simulink model "heatdrive_ecc_coupled_se21"  (R2025b)
settings: Solver=ode23t  StartTime=0.0  StopTime=10  FixedStep=0.1  MaxStep=0.4  RelTol=1e-2  AbsTol=1e-3
values from neighbouring files (symbols this model uses):
  cold_load_heat_W = 0.0    (= 0)    [Build_Simulink_Exchange_Params.m]
  cold_load_T_init = get_stage_field(stage_config, 'cold_load_T_in', get_stage_field(stage_config,          'chip_T_in', get_option_field(exchange_options, 'cold_load_T_init', get_option_field(exchange_options, 'chip_T_init', 293.0))))    [Build_Simulink_Exchange_Params.m]    (also in Create_Simulink_Exchange_Runtime.m = get_option_field(options, 'cold_load_T_init',          get_o)
  cold_sink_T_init = get_stage_field(stage_config, 'cold_sink_T_in', get_option_field(exchange_options, 'cold_sink_T_init', 293.0))    [Build_Simulink_Exchange_Params.m]    (also in Create_Simulink_Exchange_Runtime.m = get_option_field(options, 'cold_sink_T_init', ambient_T_init)
  hot_sink_T_init = get_stage_field(stage_config, 'hot_sink_T_in', get_option_field(exchange_options, 'hot_sink_T_init', 293.0))    [Build_Simulink_Exchange_Params.m]    (also in Create_Simulink_Exchange_Runtime.m = get_option_field(options, 'hot_sink_T_init', ambient_T_init))
  mdot_cooldown_source_kgps = mdot_target_kgps    [Build_Simulink_Exchange_Params.m]
  mdot_hold_source_kgps = mdot_target_kgps    [Build_Simulink_Exchange_Params.m]
  pressure_pi_bias_MPa = pressure_pi_dp_guess_MPa    [Build_Simulink_Exchange_Params.m]
  pressure_pi_error_filter_tau_s = max(get_option_field(exchange_options, 'pressure_pi_error_filter_tau_s', 0.002), 1.0e-5)    [Build_Simulink_Exchange_Params.m]
  pressure_pi_error_normalization_gain_kgps_inv = 1.0    (= 1)    [Build_Simulink_Exchange_Params.m]
  pressure_pi_max_MPa = pressure_pi_dp_guess_MPa + pressure_pi_margin_MPa    [Build_Simulink_Exchange_Params.m]
  shex_sink_T_init = get_option_field(exchange_options, 'shex_sink_T_init', hot_sink_T_init)    [Build_Simulink_Exchange_Params.m]
undefined symbols (not defined in the file or in its folder): constitutive_sample_time_s, constitutive_state21_initial, se_constitutive_T21_initial, se_pressure_integrator_max_MPa, se_pressure_pi_ki_MPa_per_kgps_s, se_pressure_pi_kp_MPa_per_kgps, se_pressure_pi_min_MPa, se_solver_T_init_21_internal, se_stage2_pressure_integrator_min_MPa, se_stage4_pressure_integrator_min_MPa, sma_constitutive_T21_initial, sma_mdot_stage1_source_kgps, sma_mdot_stage3_source_kgps, sma_pressure_integrator_max_MPa, sma_pressure_integrator_min_MPa, sma_pressure_pi_ki_MPa_per_kgps_s, sma_pressure_pi_kp_MPa_per_kgps, sma_pressure_pi_min_MPa, sma_solver_T_init_21_internal
libraries: fl_lib x484, nesl_utility x232, SimscapeFluids_lib x20
(part 2 of 8)

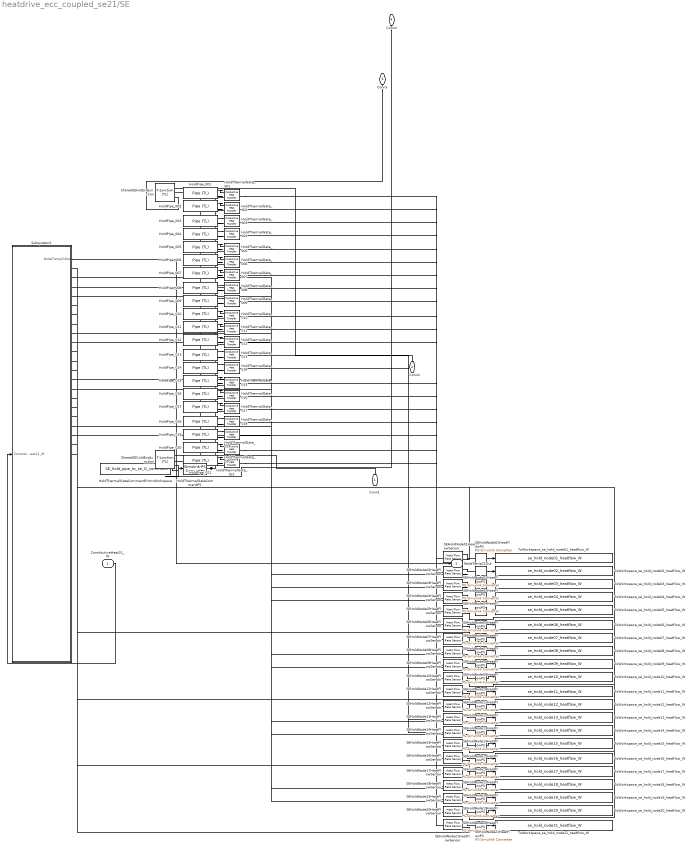
== system heatdrive_ecc_coupled_se21/SE ==
  ConstitutiveHeat21_W : Inport
  HoldPipe_001 : fl_lib/Thermal Liquid/Elements/Pipe (TL)  length=se_article_pipe_segment_l m  area=se_article_pipe_fa m^2  Dh=se_article_pipe_Dh m  length_add=0 m  roughness=15e-6 m  Re_lam=2000  Re_tur=4000  shape_factor=64  Nu_lam=se_article_Nu  dynamic_compressibility=false  inertia=false  p0=1 MPa  T0=se_hold_fluid_T_init K  mdot0=0 kg/s  p_nominal=1 MPa  T_nominal=293.15 K
  HoldPipe_002 : fl_lib/Thermal Liquid/Elements/Pipe (TL)  length=se_article_pipe_segment_l m  area=se_article_pipe_fa m^2  Dh=se_article_pipe_Dh m  length_add=0 m  roughness=15e-6 m  Re_lam=2000  Re_tur=4000  shape_factor=64  Nu_lam=se_article_Nu  dynamic_compressibility=false  inertia=false  p0=1 MPa  T0=se_hold_fluid_T_init K  mdot0=0 kg/s  p_nominal=1 MPa  T_nominal=293.15 K
  HoldPipe_003 : fl_lib/Thermal Liquid/Elements/Pipe (TL)  length=se_article_pipe_segment_l m  area=se_article_pipe_fa m^2  Dh=se_article_pipe_Dh m  length_add=0 m  roughness=15e-6 m  Re_lam=2000  Re_tur=4000  shape_factor=64  Nu_lam=se_article_Nu  dynamic_compressibility=false  inertia=false  p0=1 MPa  T0=se_hold_fluid_T_init K  mdot0=0 kg/s  p_nominal=1 MPa  T_nominal=293.15 K
  HoldPipe_004 : fl_lib/Thermal Liquid/Elements/Pipe (TL)  length=se_article_pipe_segment_l m  area=se_article_pipe_fa m^2  Dh=se_article_pipe_Dh m  length_add=0 m  roughness=15e-6 m  Re_lam=2000  Re_tur=4000  shape_factor=64  Nu_lam=se_article_Nu  dynamic_compressibility=false  inertia=false  p0=1 MPa  T0=se_hold_fluid_T_init K  mdot0=0 kg/s  p_nominal=1 MPa  T_nominal=293.15 K
  HoldPipe_005 : fl_lib/Thermal Liquid/Elements/Pipe (TL)  length=se_article_pipe_segment_l m  area=se_article_pipe_fa m^2  Dh=se_article_pipe_Dh m  length_add=0 m  roughness=15e-6 m  Re_lam=2000  Re_tur=4000  shape_factor=64  Nu_lam=se_article_Nu  dynamic_compressibility=false  inertia=false  p0=1 MPa  T0=se_hold_fluid_T_init K  mdot0=0 kg/s  p_nominal=1 MPa  T_nominal=293.15 K
  HoldPipe_006 : fl_lib/Thermal Liquid/Elements/Pipe (TL)  length=se_article_pipe_segment_l m  area=se_article_pipe_fa m^2  Dh=se_article_pipe_Dh m  length_add=0 m  roughness=15e-6 m  Re_lam=2000  Re_tur=4000  shape_factor=64  Nu_lam=se_article_Nu  dynamic_compressibility=false  inertia=false  p0=1 MPa  T0=se_hold_fluid_T_init K  mdot0=0 kg/s  p_nominal=1 MPa  T_nominal=293.15 K
  HoldPipe_007 : fl_lib/Thermal Liquid/Elements/Pipe (TL)  length=se_article_pipe_segment_l m  area=se_article_pipe_fa m^2  Dh=se_article_pipe_Dh m  length_add=0 m  roughness=15e-6 m  Re_lam=2000  Re_tur=4000  shape_factor=64  Nu_lam=se_article_Nu  dynamic_compressibility=false  inertia=false  p0=1 MPa  T0=se_hold_fluid_T_init K  mdot0=0 kg/s  p_nominal=1 MPa  T_nominal=293.15 K
  HoldPipe_008 : fl_lib/Thermal Liquid/Elements/Pipe (TL)  length=se_article_pipe_segment_l m  area=se_article_pipe_fa m^2  Dh=se_article_pipe_Dh m  length_add=0 m  roughness=15e-6 m  Re_lam=2000  Re_tur=4000  shape_factor=64  Nu_lam=se_article_Nu  dynamic_compressibility=false  inertia=false  p0=1 MPa  T0=se_hold_fluid_T_init K  mdot0=0 kg/s  p_nominal=1 MPa  T_nominal=293.15 K
  HoldPipe_009 : fl_lib/Thermal Liquid/Elements/Pipe (TL)  length=se_article_pipe_segment_l m  area=se_article_pipe_fa m^2  Dh=se_article_pipe_Dh m  length_add=0 m  roughness=15e-6 m  Re_lam=2000  Re_tur=4000  shape_factor=64  Nu_lam=se_article_Nu  dynamic_compressibility=false  inertia=false  p0=1 MPa  T0=se_hold_fluid_T_init K  mdot0=0 kg/s  p_nominal=1 MPa  T_nominal=293.15 K
  HoldPipe_010 : fl_lib/Thermal Liquid/Elements/Pipe (TL)  length=se_article_pipe_segment_l m  area=se_article_pipe_fa m^2  Dh=se_article_pipe_Dh m  length_add=0 m  roughness=15e-6 m  Re_lam=2000  Re_tur=4000  shape_factor=64  Nu_lam=se_article_Nu  dynamic_compressibility=false  inertia=false  p0=1 MPa  T0=se_hold_fluid_T_init K  mdot0=0 kg/s  p_nominal=1 MPa  T_nominal=293.15 K
  HoldPipe_011 : fl_lib/Thermal Liquid/Elements/Pipe (TL)  length=se_article_pipe_segment_l m  area=se_article_pipe_fa m^2  Dh=se_article_pipe_Dh m  length_add=0 m  roughness=15e-6 m  Re_lam=2000  Re_tur=4000  shape_factor=64  Nu_lam=se_article_Nu  dynamic_compressibility=false  inertia=false  p0=1 MPa  T0=se_hold_fluid_T_init K  mdot0=0 kg/s  p_nominal=1 MPa  T_nominal=293.15 K
  HoldPipe_012 : fl_lib/Thermal Liquid/Elements/Pipe (TL)  length=se_article_pipe_segment_l m  area=se_article_pipe_fa m^2  Dh=se_article_pipe_Dh m  length_add=0 m  roughness=15e-6 m  Re_lam=2000  Re_tur=4000  shape_factor=64  Nu_lam=se_article_Nu  dynamic_compressibility=false  inertia=false  p0=1 MPa  T0=se_hold_fluid_T_init K  mdot0=0 kg/s  p_nominal=1 MPa  T_nominal=293.15 K
  HoldPipe_013 : fl_lib/Thermal Liquid/Elements/Pipe (TL)  length=se_article_pipe_segment_l m  area=se_article_pipe_fa m^2  Dh=se_article_pipe_Dh m  length_add=0 m  roughness=15e-6 m  Re_lam=2000  Re_tur=4000  shape_factor=64  Nu_lam=se_article_Nu  dynamic_compressibility=false  inertia=false  p0=1 MPa  T0=se_hold_fluid_T_init K  mdot0=0 kg/s  p_nominal=1 MPa  T_nominal=293.15 K
  HoldPipe_014 : fl_lib/Thermal Liquid/Elements/Pipe (TL)  length=se_article_pipe_segment_l m  area=se_article_pipe_fa m^2  Dh=se_article_pipe_Dh m  length_add=0 m  roughness=15e-6 m  Re_lam=2000  Re_tur=4000  shape_factor=64  Nu_lam=se_article_Nu  dynamic_compressibility=false  inertia=false  p0=1 MPa  T0=se_hold_fluid_T_init K  mdot0=0 kg/s  p_nominal=1 MPa  T_nominal=293.15 K
  HoldPipe_015 : fl_lib/Thermal Liquid/Elements/Pipe (TL)  length=se_article_pipe_segment_l m  area=se_article_pipe_fa m^2  Dh=se_article_pipe_Dh m  length_add=0 m  roughness=15e-6 m  Re_lam=2000  Re_tur=4000  shape_factor=64  Nu_lam=se_article_Nu  dynamic_compressibility=false  inertia=false  p0=1 MPa  T0=se_hold_fluid_T_init K  mdot0=0 kg/s  p_nominal=1 MPa  T_nominal=293.15 K
  HoldPipe_016 : fl_lib/Thermal Liquid/Elements/Pipe (TL)  length=se_article_pipe_segment_l m  area=se_article_pipe_fa m^2  Dh=se_article_pipe_Dh m  length_add=0 m  roughness=15e-6 m  Re_lam=2000  Re_tur=4000  shape_factor=64  Nu_lam=se_article_Nu  dynamic_compressibility=false  inertia=false  p0=1 MPa  T0=se_hold_fluid_T_init K  mdot0=0 kg/s  p_nominal=1 MPa  T_nominal=293.15 K
  HoldPipe_017 : fl_lib/Thermal Liquid/Elements/Pipe (TL)  length=se_article_pipe_segment_l m  area=se_article_pipe_fa m^2  Dh=se_article_pipe_Dh m  length_add=0 m  roughness=15e-6 m  Re_lam=2000  Re_tur=4000  shape_factor=64  Nu_lam=se_article_Nu  dynamic_compressibility=false  inertia=false  p0=1 MPa  T0=se_hold_fluid_T_init K  mdot0=0 kg/s  p_nominal=1 MPa  T_nominal=293.15 K
  HoldPipe_018 : fl_lib/Thermal Liquid/Elements/Pipe (TL)  length=se_article_pipe_segment_l m  area=se_article_pipe_fa m^2  Dh=se_article_pipe_Dh m  length_add=0 m  roughness=15e-6 m  Re_lam=2000  Re_tur=4000  shape_factor=64  Nu_lam=se_article_Nu  dynamic_compressibility=false  inertia=false  p0=1 MPa  T0=se_hold_fluid_T_init K  mdot0=0 kg/s  p_nominal=1 MPa  T_nominal=293.15 K
  HoldPipe_019 : fl_lib/Thermal Liquid/Elements/Pipe (TL)  length=se_article_pipe_segment_l m  area=se_article_pipe_fa m^2  Dh=se_article_pipe_Dh m  length_add=0 m  roughness=15e-6 m  Re_lam=2000  Re_tur=4000  shape_factor=64  Nu_lam=se_article_Nu  dynamic_compressibility=false  inertia=false  p0=1 MPa  T0=se_hold_fluid_T_init K  mdot0=0 kg/s  p_nominal=1 MPa  T_nominal=293.15 K
  HoldPipe_020 : fl_lib/Thermal Liquid/Elements/Pipe (TL)  length=se_article_pipe_segment_l m  area=se_article_pipe_fa m^2  Dh=se_article_pipe_Dh m  length_add=0 m  roughness=15e-6 m  Re_lam=2000  Re_tur=4000  shape_factor=64  Nu_lam=se_article_Nu  dynamic_compressibility=false  inertia=false  p0=1 MPa  T0=se_hold_fluid_T_init K  mdot0=0 kg/s  p_nominal=1 MPa  T_nominal=293.15 K
  HoldPipe_021 : fl_lib/Thermal Liquid/Elements/Pipe (TL)  length=se_article_pipe_segment_l m  area=se_article_pipe_fa m^2  Dh=se_article_pipe_Dh m  length_add=0 m  roughness=15e-6 m  Re_lam=2000  Re_tur=4000  shape_factor=64  Nu_lam=se_article_Nu  dynamic_compressibility=false  inertia=false  p0=1 MPa  T0=se_hold_fluid_T_init K  mdot0=0 kg/s  p_nominal=1 MPa  T_nominal=293.15 K
  HoldThermalGateCommandFromWorkspace : FromWorkspace  VariableName=SE_hold_pipe_to_se_G_command  Interpolate=off  OutputAfterFinalValue=Holding final value
  HoldThermalGateCommandPS : nesl_utility/Simulink-PS Converter  PhysicalDomain=network_engine_domain  SubClassName=ps_input  LeftPortType=input  RightPortType=output  PseudoPeriodic=off  Frequencies=[]  NoiseDistribution=none  NoiseParameters=[]  Unit=W/(K*m)  AffineConversion=off  FilteringAndDerivatives=provide  SimscapeFilterOrder=1  InputFilterTimeConstant=0.001  UdotUserProvided=0
  HoldThermalGate_001 : fl_lib/Thermal/Thermal Elements/Conductive Heat Transfer  thermal_type=foundation.enum.ConstantVariableTabulated.Variable  wall_geometry=foundation.enum.ConductionWallGeometry.Planar  area=1 m^2  thickness=1 m  d_in=0.05 m  d_out=0.1 m  L=1 m  th_cond_min=thermal_gate_min_conductivity_W_per_mK W/(K*m)  th_cond=sma_hold_pipe_to_sma_G_W_per_K W/(K*m)  th_cond_TLU=[413, 401, 392, 383, 371, 357, 342] W/(K*m)  temp_TLU=[200, 273, 400, 600, 800, 1000, 1200] K  T_specify=off  T_priority=None  T=0 K  T_nominal_specify=off  T_nominal_value=1  T_nominal_unit=K  Q_specify=off  Q_priority=None  Q=0 W  Q_nominal_specify=off  Q_nominal_value=1  Q_nominal_unit=W
      settings: InternalSimscapePortConfiguration="{\"Bottom\":[],\"Left\":[{\"id\":\"A\",\"label\":\"A\",\"type\":\"foundation.thermal.thermal\"},{\"id\":\"var_th_cond\",\"label\":\"K\",\"type\":\"input\"}],\"Right\":[{\"id\":\"B\",\"label\":\"B\",\"type\":\"foundation.thermal.thermal\"}],\"Top\":[]}"
  HoldThermalGate_002 : fl_lib/Thermal/Thermal Elements/Conductive Heat Transfer  thermal_type=foundation.enum.ConstantVariableTabulated.Variable  wall_geometry=foundation.enum.ConductionWallGeometry.Planar  area=1 m^2  thickness=1 m  d_in=0.05 m  d_out=0.1 m  L=1 m  th_cond_min=thermal_gate_min_conductivity_W_per_mK W/(K*m)  th_cond=sma_hold_pipe_to_sma_G_W_per_K W/(K*m)  th_cond_TLU=[413, 401, 392, 383, 371, 357, 342] W/(K*m)  temp_TLU=[200, 273, 400, 600, 800, 1000, 1200] K  T_specify=off  T_priority=None  T=0 K  T_nominal_specify=off  T_nominal_value=1  T_nominal_unit=K  Q_specify=off  Q_priority=None  Q=0 W  Q_nominal_specify=off  Q_nominal_value=1  Q_nominal_unit=W
      settings: InternalSimscapePortConfiguration="{\"Bottom\":[],\"Left\":[{\"id\":\"A\",\"label\":\"A\",\"type\":\"foundation.thermal.thermal\"},{\"id\":\"var_th_cond\",\"label\":\"K\",\"type\":\"input\"}],\"Right\":[{\"id\":\"B\",\"label\":\"B\",\"type\":\"foundation.thermal.thermal\"}],\"Top\":[]}"
  HoldThermalGate_003 : fl_lib/Thermal/Thermal Elements/Conductive Heat Transfer  thermal_type=foundation.enum.ConstantVariableTabulated.Variable  wall_geometry=foundation.enum.ConductionWallGeometry.Planar  area=1 m^2  thickness=1 m  d_in=0.05 m  d_out=0.1 m  L=1 m  th_cond_min=thermal_gate_min_conductivity_W_per_mK W/(K*m)  th_cond=sma_hold_pipe_to_sma_G_W_per_K W/(K*m)  th_cond_TLU=[413, 401, 392, 383, 371, 357, 342] W/(K*m)  temp_TLU=[200, 273, 400, 600, 800, 1000, 1200] K  T_specify=off  T_priority=None  T=0 K  T_nominal_specify=off  T_nominal_value=1  T_nominal_unit=K  Q_specify=off  Q_priority=None  Q=0 W  Q_nominal_specify=off  Q_nominal_value=1  Q_nominal_unit=W
      settings: InternalSimscapePortConfiguration="{\"Bottom\":[],\"Left\":[{\"id\":\"A\",\"label\":\"A\",\"type\":\"foundation.thermal.thermal\"},{\"id\":\"var_th_cond\",\"label\":\"K\",\"type\":\"input\"}],\"Right\":[{\"id\":\"B\",\"label\":\"B\",\"type\":\"foundation.thermal.thermal\"}],\"Top\":[]}"
  HoldThermalGate_004 : fl_lib/Thermal/Thermal Elements/Conductive Heat Transfer  thermal_type=foundation.enum.ConstantVariableTabulated.Variable  wall_geometry=foundation.enum.ConductionWallGeometry.Planar  area=1 m^2  thickness=1 m  d_in=0.05 m  d_out=0.1 m  L=1 m  th_cond_min=thermal_gate_min_conductivity_W_per_mK W/(K*m)  th_cond=sma_hold_pipe_to_sma_G_W_per_K W/(K*m)  th_cond_TLU=[413, 401, 392, 383, 371, 357, 342] W/(K*m)  temp_TLU=[200, 273, 400, 600, 800, 1000, 1200] K  T_specify=off  T_priority=None  T=0 K  T_nominal_specify=off  T_nominal_value=1  T_nominal_unit=K  Q_specify=off  Q_priority=None  Q=0 W  Q_nominal_specify=off  Q_nominal_value=1  Q_nominal_unit=W
      settings: InternalSimscapePortConfiguration="{\"Bottom\":[],\"Left\":[{\"id\":\"A\",\"label\":\"A\",\"type\":\"foundation.thermal.thermal\"},{\"id\":\"var_th_cond\",\"label\":\"K\",\"type\":\"input\"}],\"Right\":[{\"id\":\"B\",\"label\":\"B\",\"type\":\"foundation.thermal.thermal\"}],\"Top\":[]}"
  HoldThermalGate_005 : fl_lib/Thermal/Thermal Elements/Conductive Heat Transfer  thermal_type=foundation.enum.ConstantVariableTabulated.Variable  wall_geometry=foundation.enum.ConductionWallGeometry.Planar  area=1 m^2  thickness=1 m  d_in=0.05 m  d_out=0.1 m  L=1 m  th_cond_min=thermal_gate_min_conductivity_W_per_mK W/(K*m)  th_cond=sma_hold_pipe_to_sma_G_W_per_K W/(K*m)  th_cond_TLU=[413, 401, 392, 383, 371, 357, 342] W/(K*m)  temp_TLU=[200, 273, 400, 600, 800, 1000, 1200] K  T_specify=off  T_priority=None  T=0 K  T_nominal_specify=off  T_nominal_value=1  T_nominal_unit=K  Q_specify=off  Q_priority=None  Q=0 W  Q_nominal_specify=off  Q_nominal_value=1  Q_nominal_unit=W
      settings: InternalSimscapePortConfiguration="{\"Bottom\":[],\"Left\":[{\"id\":\"A\",\"label\":\"A\",\"type\":\"foundation.thermal.thermal\"},{\"id\":\"var_th_cond\",\"label\":\"K\",\"type\":\"input\"}],\"Right\":[{\"id\":\"B\",\"label\":\"B\",\"type\":\"foundation.thermal.thermal\"}],\"Top\":[]}"
  HoldThermalGate_006 : fl_lib/Thermal/Thermal Elements/Conductive Heat Transfer  thermal_type=foundation.enum.ConstantVariableTabulated.Variable  wall_geometry=foundation.enum.ConductionWallGeometry.Planar  area=1 m^2  thickness=1 m  d_in=0.05 m  d_out=0.1 m  L=1 m  th_cond_min=thermal_gate_min_conductivity_W_per_mK W/(K*m)  th_cond=sma_hold_pipe_to_sma_G_W_per_K W/(K*m)  th_cond_TLU=[413, 401, 392, 383, 371, 357, 342] W/(K*m)  temp_TLU=[200, 273, 400, 600, 800, 1000, 1200] K  T_specify=off  T_priority=None  T=0 K  T_nominal_specify=off  T_nominal_value=1  T_nominal_unit=K  Q_specify=off  Q_priority=None  Q=0 W  Q_nominal_specify=off  Q_nominal_value=1  Q_nominal_unit=W
      settings: InternalSimscapePortConfiguration="{\"Bottom\":[],\"Left\":[{\"id\":\"A\",\"label\":\"A\",\"type\":\"foundation.thermal.thermal\"},{\"id\":\"var_th_cond\",\"label\":\"K\",\"type\":\"input\"}],\"Right\":[{\"id\":\"B\",\"label\":\"B\",\"type\":\"foundation.thermal.thermal\"}],\"Top\":[]}"
  HoldThermalGate_007 : fl_lib/Thermal/Thermal Elements/Conductive Heat Transfer  thermal_type=foundation.enum.ConstantVariableTabulated.Variable  wall_geometry=foundation.enum.ConductionWallGeometry.Planar  area=1 m^2  thickness=1 m  d_in=0.05 m  d_out=0.1 m  L=1 m  th_cond_min=thermal_gate_min_conductivity_W_per_mK W/(K*m)  th_cond=sma_hold_pipe_to_sma_G_W_per_K W/(K*m)  th_cond_TLU=[413, 401, 392, 383, 371, 357, 342] W/(K*m)  temp_TLU=[200, 273, 400, 600, 800, 1000, 1200] K  T_specify=off  T_priority=None  T=0 K  T_nominal_specify=off  T_nominal_value=1  T_nominal_unit=K  Q_specify=off  Q_priority=None  Q=0 W  Q_nominal_specify=off  Q_nominal_value=1  Q_nominal_unit=W
      settings: InternalSimscapePortConfiguration="{\"Bottom\":[],\"Left\":[{\"id\":\"A\",\"label\":\"A\",\"type\":\"foundation.thermal.thermal\"},{\"id\":\"var_th_cond\",\"label\":\"K\",\"type\":\"input\"}],\"Right\":[{\"id\":\"B\",\"label\":\"B\",\"type\":\"foundation.thermal.thermal\"}],\"Top\":[]}"
  HoldThermalGate_008 : fl_lib/Thermal/Thermal Elements/Conductive Heat Transfer  thermal_type=foundation.enum.ConstantVariableTabulated.Variable  wall_geometry=foundation.enum.ConductionWallGeometry.Planar  area=1 m^2  thickness=1 m  d_in=0.05 m  d_out=0.1 m  L=1 m  th_cond_min=thermal_gate_min_conductivity_W_per_mK W/(K*m)  th_cond=sma_hold_pipe_to_sma_G_W_per_K W/(K*m)  th_cond_TLU=[413, 401, 392, 383, 371, 357, 342] W/(K*m)  temp_TLU=[200, 273, 400, 600, 800, 1000, 1200] K  T_specify=off  T_priority=None  T=0 K  T_nominal_specify=off  T_nominal_value=1  T_nominal_unit=K  Q_specify=off  Q_priority=None  Q=0 W  Q_nominal_specify=off  Q_nominal_value=1  Q_nominal_unit=W
      settings: InternalSimscapePortConfiguration="{\"Bottom\":[],\"Left\":[{\"id\":\"A\",\"label\":\"A\",\"type\":\"foundation.thermal.thermal\"},{\"id\":\"var_th_cond\",\"label\":\"K\",\"type\":\"input\"}],\"Right\":[{\"id\":\"B\",\"label\":\"B\",\"type\":\"foundation.thermal.thermal\"}],\"Top\":[]}"
  HoldThermalGate_009 : fl_lib/Thermal/Thermal Elements/Conductive Heat Transfer  thermal_type=foundation.enum.ConstantVariableTabulated.Variable  wall_geometry=foundation.enum.ConductionWallGeometry.Planar  area=1 m^2  thickness=1 m  d_in=0.05 m  d_out=0.1 m  L=1 m  th_cond_min=thermal_gate_min_conductivity_W_per_mK W/(K*m)  th_cond=sma_hold_pipe_to_sma_G_W_per_K W/(K*m)  th_cond_TLU=[413, 401, 392, 383, 371, 357, 342] W/(K*m)  temp_TLU=[200, 273, 400, 600, 800, 1000, 1200] K  T_specify=off  T_priority=None  T=0 K  T_nominal_specify=off  T_nominal_value=1  T_nominal_unit=K  Q_specify=off  Q_priority=None  Q=0 W  Q_nominal_specify=off  Q_nominal_value=1  Q_nominal_unit=W
      settings: InternalSimscapePortConfiguration="{\"Bottom\":[],\"Left\":[{\"id\":\"A\",\"label\":\"A\",\"type\":\"foundation.thermal.thermal\"},{\"id\":\"var_th_cond\",\"label\":\"K\",\"type\":\"input\"}],\"Right\":[{\"id\":\"B\",\"label\":\"B\",\"type\":\"foundation.thermal.thermal\"}],\"Top\":[]}"
  HoldThermalGate_010 : fl_lib/Thermal/Thermal Elements/Conductive Heat Transfer  thermal_type=foundation.enum.ConstantVariableTabulated.Variable  wall_geometry=foundation.enum.ConductionWallGeometry.Planar  area=1 m^2  thickness=1 m  d_in=0.05 m  d_out=0.1 m  L=1 m  th_cond_min=thermal_gate_min_conductivity_W_per_mK W/(K*m)  th_cond=sma_hold_pipe_to_sma_G_W_per_K W/(K*m)  th_cond_TLU=[413, 401, 392, 383, 371, 357, 342] W/(K*m)  temp_TLU=[200, 273, 400, 600, 800, 1000, 1200] K  T_specify=off  T_priority=None  T=0 K  T_nominal_specify=off  T_nominal_value=1  T_nominal_unit=K  Q_specify=off  Q_priority=None  Q=0 W  Q_nominal_specify=off  Q_nominal_value=1  Q_nominal_unit=W
      settings: InternalSimscapePortConfiguration="{\"Bottom\":[],\"Left\":[{\"id\":\"A\",\"label\":\"A\",\"type\":\"foundation.thermal.thermal\"},{\"id\":\"var_th_cond\",\"label\":\"K\",\"type\":\"input\"}],\"Right\":[{\"id\":\"B\",\"label\":\"B\",\"type\":\"foundation.thermal.thermal\"}],\"Top\":[]}"
  HoldThermalGate_011 : fl_lib/Thermal/Thermal Elements/Conductive Heat Transfer  thermal_type=foundation.enum.ConstantVariableTabulated.Variable  wall_geometry=foundation.enum.ConductionWallGeometry.Planar  area=1 m^2  thickness=1 m  d_in=0.05 m  d_out=0.1 m  L=1 m  th_cond_min=thermal_gate_min_conductivity_W_per_mK W/(K*m)  th_cond=sma_hold_pipe_to_sma_G_W_per_K W/(K*m)  th_cond_TLU=[413, 401, 392, 383, 371, 357, 342] W/(K*m)  temp_TLU=[200, 273, 400, 600, 800, 1000, 1200] K  T_specify=off  T_priority=None  T=0 K  T_nominal_specify=off  T_nominal_value=1  T_nominal_unit=K  Q_specify=off  Q_priority=None  Q=0 W  Q_nominal_specify=off  Q_nominal_value=1  Q_nominal_unit=W
      settings: InternalSimscapePortConfiguration="{\"Bottom\":[],\"Left\":[{\"id\":\"A\",\"label\":\"A\",\"type\":\"foundation.thermal.thermal\"},{\"id\":\"var_th_cond\",\"label\":\"K\",\"type\":\"input\"}],\"Right\":[{\"id\":\"B\",\"label\":\"B\",\"type\":\"foundation.thermal.thermal\"}],\"Top\":[]}"
  HoldThermalGate_012 : fl_lib/Thermal/Thermal Elements/Conductive Heat Transfer  thermal_type=foundation.enum.ConstantVariableTabulated.Variable  wall_geometry=foundation.enum.ConductionWallGeometry.Planar  area=1 m^2  thickness=1 m  d_in=0.05 m  d_out=0.1 m  L=1 m  th_cond_min=thermal_gate_min_conductivity_W_per_mK W/(K*m)  th_cond=sma_hold_pipe_to_sma_G_W_per_K W/(K*m)  th_cond_TLU=[413, 401, 392, 383, 371, 357, 342] W/(K*m)  temp_TLU=[200, 273, 400, 600, 800, 1000, 1200] K  T_specify=off  T_priority=None  T=0 K  T_nominal_specify=off  T_nominal_value=1  T_nominal_unit=K  Q_specify=off  Q_priority=None  Q=0 W  Q_nominal_specify=off  Q_nominal_value=1  Q_nominal_unit=W
      settings: InternalSimscapePortConfiguration="{\"Bottom\":[],\"Left\":[{\"id\":\"A\",\"label\":\"A\",\"type\":\"foundation.thermal.thermal\"},{\"id\":\"var_th_cond\",\"label\":\"K\",\"type\":\"input\"}],\"Right\":[{\"id\":\"B\",\"label\":\"B\",\"type\":\"foundation.thermal.thermal\"}],\"Top\":[]}"
  HoldThermalGate_013 : fl_lib/Thermal/Thermal Elements/Conductive Heat Transfer  thermal_type=foundation.enum.ConstantVariableTabulated.Variable  wall_geometry=foundation.enum.ConductionWallGeometry.Planar  area=1 m^2  thickness=1 m  d_in=0.05 m  d_out=0.1 m  L=1 m  th_cond_min=thermal_gate_min_conductivity_W_per_mK W/(K*m)  th_cond=sma_hold_pipe_to_sma_G_W_per_K W/(K*m)  th_cond_TLU=[413, 401, 392, 383, 371, 357, 342] W/(K*m)  temp_TLU=[200, 273, 400, 600, 800, 1000, 1200] K  T_specify=off  T_priority=None  T=0 K  T_nominal_specify=off  T_nominal_value=1  T_nominal_unit=K  Q_specify=off  Q_priority=None  Q=0 W  Q_nominal_specify=off  Q_nominal_value=1  Q_nominal_unit=W
      settings: InternalSimscapePortConfiguration="{\"Bottom\":[],\"Left\":[{\"id\":\"A\",\"label\":\"A\",\"type\":\"foundation.thermal.thermal\"},{\"id\":\"var_th_cond\",\"label\":\"K\",\"type\":\"input\"}],\"Right\":[{\"id\":\"B\",\"label\":\"B\",\"type\":\"foundation.thermal.thermal\"}],\"Top\":[]}"
  HoldThermalGate_014 : fl_lib/Thermal/Thermal Elements/Conductive Heat Transfer  thermal_type=foundation.enum.ConstantVariableTabulated.Variable  wall_geometry=foundation.enum.ConductionWallGeometry.Planar  area=1 m^2  thickness=1 m  d_in=0.05 m  d_out=0.1 m  L=1 m  th_cond_min=thermal_gate_min_conductivity_W_per_mK W/(K*m)  th_cond=sma_hold_pipe_to_sma_G_W_per_K W/(K*m)  th_cond_TLU=[413, 401, 392, 383, 371, 357, 342] W/(K*m)  temp_TLU=[200, 273, 400, 600, 800, 1000, 1200] K  T_specify=off  T_priority=None  T=0 K  T_nominal_specify=off  T_nominal_value=1  T_nominal_unit=K  Q_specify=off  Q_priority=None  Q=0 W  Q_nominal_specify=off  Q_nominal_value=1  Q_nominal_unit=W
      settings: InternalSimscapePortConfiguration="{\"Bottom\":[],\"Left\":[{\"id\":\"A\",\"label\":\"A\",\"type\":\"foundation.thermal.thermal\"},{\"id\":\"var_th_cond\",\"label\":\"K\",\"type\":\"input\"}],\"Right\":[{\"id\":\"B\",\"label\":\"B\",\"type\":\"foundation.thermal.thermal\"}],\"Top\":[]}"
  HoldThermalGate_015 : fl_lib/Thermal/Thermal Elements/Conductive Heat Transfer  thermal_type=foundation.enum.ConstantVariableTabulated.Variable  wall_geometry=foundation.enum.ConductionWallGeometry.Planar  area=1 m^2  thickness=1 m  d_in=0.05 m  d_out=0.1 m  L=1 m  th_cond_min=thermal_gate_min_conductivity_W_per_mK W/(K*m)  th_cond=sma_hold_pipe_to_sma_G_W_per_K W/(K*m)  th_cond_TLU=[413, 401, 392, 383, 371, 357, 342] W/(K*m)  temp_TLU=[200, 273, 400, 600, 800, 1000, 1200] K  T_specify=off  T_priority=None  T=0 K  T_nominal_specify=off  T_nominal_value=1  T_nominal_unit=K  Q_specify=off  Q_priority=None  Q=0 W  Q_nominal_specify=off  Q_nominal_value=1  Q_nominal_unit=W
      settings: InternalSimscapePortConfiguration="{\"Bottom\":[],\"Left\":[{\"id\":\"A\",\"label\":\"A\",\"type\":\"foundation.thermal.thermal\"},{\"id\":\"var_th_cond\",\"label\":\"K\",\"type\":\"input\"}],\"Right\":[{\"id\":\"B\",\"label\":\"B\",\"type\":\"foundation.thermal.thermal\"}],\"Top\":[]}"
  HoldThermalGate_016 : fl_lib/Thermal/Thermal Elements/Conductive Heat Transfer  thermal_type=foundation.enum.ConstantVariableTabulated.Variable  wall_geometry=foundation.enum.ConductionWallGeometry.Planar  area=1 m^2  thickness=1 m  d_in=0.05 m  d_out=0.1 m  L=1 m  th_cond_min=thermal_gate_min_conductivity_W_per_mK W/(K*m)  th_cond=sma_hold_pipe_to_sma_G_W_per_K W/(K*m)  th_cond_TLU=[413, 401, 392, 383, 371, 357, 342] W/(K*m)  temp_TLU=[200, 273, 400, 600, 800, 1000, 1200] K  T_specify=off  T_priority=None  T=0 K  T_nominal_specify=off  T_nominal_value=1  T_nominal_unit=K  Q_specify=off  Q_priority=None  Q=0 W  Q_nominal_specify=off  Q_nominal_value=1  Q_nominal_unit=W
      settings: InternalSimscapePortConfiguration="{\"Bottom\":[],\"Left\":[{\"id\":\"A\",\"label\":\"A\",\"type\":\"foundation.thermal.thermal\"},{\"id\":\"var_th_cond\",\"label\":\"K\",\"type\":\"input\"}],\"Right\":[{\"id\":\"B\",\"label\":\"B\",\"type\":\"foundation.thermal.thermal\"}],\"Top\":[]}"
  HoldThermalGate_017 : fl_lib/Thermal/Thermal Elements/Conductive Heat Transfer  thermal_type=foundation.enum.ConstantVariableTabulated.Variable  wall_geometry=foundation.enum.ConductionWallGeometry.Planar  area=1 m^2  thickness=1 m  d_in=0.05 m  d_out=0.1 m  L=1 m  th_cond_min=thermal_gate_min_conductivity_W_per_mK W/(K*m)  th_cond=sma_hold_pipe_to_sma_G_W_per_K W/(K*m)  th_cond_TLU=[413, 401, 392, 383, 371, 357, 342] W/(K*m)  temp_TLU=[200, 273, 400, 600, 800, 1000, 1200] K  T_specify=off  T_priority=None  T=0 K  T_nominal_specify=off  T_nominal_value=1  T_nominal_unit=K  Q_specify=off  Q_priority=None  Q=0 W  Q_nominal_specify=off  Q_nominal_value=1  Q_nominal_unit=W
      settings: InternalSimscapePortConfiguration="{\"Bottom\":[],\"Left\":[{\"id\":\"A\",\"label\":\"A\",\"type\":\"foundation.thermal.thermal\"},{\"id\":\"var_th_cond\",\"label\":\"K\",\"type\":\"input\"}],\"Right\":[{\"id\":\"B\",\"label\":\"B\",\"type\":\"foundation.thermal.thermal\"}],\"Top\":[]}"
  HoldThermalGate_018 : fl_lib/Thermal/Thermal Elements/Conductive Heat Transfer  thermal_type=foundation.enum.ConstantVariableTabulated.Variable  wall_geometry=foundation.enum.ConductionWallGeometry.Planar  area=1 m^2  thickness=1 m  d_in=0.05 m  d_out=0.1 m  L=1 m  th_cond_min=thermal_gate_min_conductivity_W_per_mK W/(K*m)  th_cond=sma_hold_pipe_to_sma_G_W_per_K W/(K*m)  th_cond_TLU=[413, 401, 392, 383, 371, 357, 342] W/(K*m)  temp_TLU=[200, 273, 400, 600, 800, 1000, 1200] K  T_specify=off  T_priority=None  T=0 K  T_nominal_specify=off  T_nominal_value=1  T_nominal_unit=K  Q_specify=off  Q_priority=None  Q=0 W  Q_nominal_specify=off  Q_nominal_value=1  Q_nominal_unit=W
      settings: InternalSimscapePortConfiguration="{\"Bottom\":[],\"Left\":[{\"id\":\"A\",\"label\":\"A\",\"type\":\"foundation.thermal.thermal\"},{\"id\":\"var_th_cond\",\"label\":\"K\",\"type\":\"input\"}],\"Right\":[{\"id\":\"B\",\"label\":\"B\",\"type\":\"foundation.thermal.thermal\"}],\"Top\":[]}"
  HoldThermalGate_019 : fl_lib/Thermal/Thermal Elements/Conductive Heat Transfer  thermal_type=foundation.enum.ConstantVariableTabulated.Variable  wall_geometry=foundation.enum.ConductionWallGeometry.Planar  area=1 m^2  thickness=1 m  d_in=0.05 m  d_out=0.1 m  L=1 m  th_cond_min=thermal_gate_min_conductivity_W_per_mK W/(K*m)  th_cond=sma_hold_pipe_to_sma_G_W_per_K W/(K*m)  th_cond_TLU=[413, 401, 392, 383, 371, 357, 342] W/(K*m)  temp_TLU=[200, 273, 400, 600, 800, 1000, 1200] K  T_specify=off  T_priority=None  T=0 K  T_nominal_specify=off  T_nominal_value=1  T_nominal_unit=K  Q_specify=off  Q_priority=None  Q=0 W  Q_nominal_specify=off  Q_nominal_value=1  Q_nominal_unit=W
      settings: InternalSimscapePortConfiguration="{\"Bottom\":[],\"Left\":[{\"id\":\"A\",\"label\":\"A\",\"type\":\"foundation.thermal.thermal\"},{\"id\":\"var_th_cond\",\"label\":\"K\",\"type\":\"input\"}],\"Right\":[{\"id\":\"B\",\"label\":\"B\",\"type\":\"foundation.thermal.thermal\"}],\"Top\":[]}"
  HoldThermalGate_020 : fl_lib/Thermal/Thermal Elements/Conductive Heat Transfer  thermal_type=foundation.enum.ConstantVariableTabulated.Variable  wall_geometry=foundation.enum.ConductionWallGeometry.Planar  area=1 m^2  thickness=1 m  d_in=0.05 m  d_out=0.1 m  L=1 m  th_cond_min=thermal_gate_min_conductivity_W_per_mK W/(K*m)  th_cond=sma_hold_pipe_to_sma_G_W_per_K W/(K*m)  th_cond_TLU=[413, 401, 392, 383, 371, 357, 342] W/(K*m)  temp_TLU=[200, 273, 400, 600, 800, 1000, 1200] K  T_specify=off  T_priority=None  T=0 K  T_nominal_specify=off  T_nominal_value=1  T_nominal_unit=K  Q_specify=off  Q_priority=None  Q=0 W  Q_nominal_specify=off  Q_nominal_value=1  Q_nominal_unit=W
      settings: InternalSimscapePortConfiguration="{\"Bottom\":[],\"Left\":[{\"id\":\"A\",\"label\":\"A\",\"type\":\"foundation.thermal.thermal\"},{\"id\":\"var_th_cond\",\"label\":\"K\",\"type\":\"input\"}],\"Right\":[{\"id\":\"B\",\"label\":\"B\",\"type\":\"foundation.thermal.thermal\"}],\"Top\":[]}"
  HoldThermalGate_021 : fl_lib/Thermal/Thermal Elements/Conductive Heat Transfer  thermal_type=foundation.enum.ConstantVariableTabulated.Variable  wall_geometry=foundation.enum.ConductionWallGeometry.Planar  area=1 m^2  thickness=1 m  d_in=0.05 m  d_out=0.1 m  L=1 m  th_cond_min=thermal_gate_min_conductivity_W_per_mK W/(K*m)  th_cond=sma_hold_pipe_to_sma_G_W_per_K W/(K*m)  th_cond_TLU=[413, 401, 392, 383, 371, 357, 342] W/(K*m)  temp_TLU=[200, 273, 400, 600, 800, 1000, 1200] K  T_specify=off  T_priority=None  T=0 K  T_nominal_specify=off  T_nominal_value=1  T_nominal_unit=K  Q_specify=off  Q_priority=None  Q=0 W  Q_nominal_specify=off  Q_nominal_value=1  Q_nominal_unit=W
      settings: InternalSimscapePortConfiguration="{\"Bottom\":[],\"Left\":[{\"id\":\"A\",\"label\":\"A\",\"type\":\"foundation.thermal.thermal\"},{\"id\":\"var_th_cond\",\"label\":\"K\",\"type\":\"input\"}],\"Right\":[{\"id\":\"B\",\"label\":\"B\",\"type\":\"foundation.thermal.thermal\"}],\"Top\":[]}"
  SEHoldNode01HeatFlowPS : nesl_utility/PS-Simulink Converter  PhysicalDomain=network_engine_domain  SubClassName=ps_output  LeftPortType=input  RightPortType=output  PseudoPeriodic=off  Frequencies=[]  VectorFormat=1-D array  Unit=W  AffineConversion=off
  SEHoldNode01HeatFlowSensor : fl_lib/Thermal/Thermal Sensors/Heat Flow Rate Sensor
  SEHoldNode02HeatFlowPS : nesl_utility/PS-Simulink Converter  PhysicalDomain=network_engine_domain  SubClassName=ps_output  LeftPortType=input  RightPortType=output  PseudoPeriodic=off  Frequencies=[]  VectorFormat=1-D array  Unit=W  AffineConversion=off
  SEHoldNode02HeatFlowSensor : fl_lib/Thermal/Thermal Sensors/Heat Flow Rate Sensor
  SEHoldNode03HeatFlowPS : nesl_utility/PS-Simulink Converter  PhysicalDomain=network_engine_domain  SubClassName=ps_output  LeftPortType=input  RightPortType=output  PseudoPeriodic=off  Frequencies=[]  VectorFormat=1-D array  Unit=W  AffineConversion=off
  SEHoldNode03HeatFlowSensor : fl_lib/Thermal/Thermal Sensors/Heat Flow Rate Sensor
  SEHoldNode04HeatFlowPS : nesl_utility/PS-Simulink Converter  PhysicalDomain=network_engine_domain  SubClassName=ps_output  LeftPortType=input  RightPortType=output  PseudoPeriodic=off  Frequencies=[]  VectorFormat=1-D array  Unit=W  AffineConversion=off
  SEHoldNode04HeatFlowSensor : fl_lib/Thermal/Thermal Sensors/Heat Flow Rate Sensor
  SEHoldNode05HeatFlowPS : nesl_utility/PS-Simulink Converter  PhysicalDomain=network_engine_domain  SubClassName=ps_output  LeftPortType=input  RightPortType=output  PseudoPeriodic=off  Frequencies=[]  VectorFormat=1-D array  Unit=W  AffineConversion=off
  SEHoldNode05HeatFlowSensor : fl_lib/Thermal/Thermal Sensors/Heat Flow Rate Sensor
  SEHoldNode06HeatFlowPS : nesl_utility/PS-Simulink Converter  PhysicalDomain=network_engine_domain  SubClassName=ps_output  LeftPortType=input  RightPortType=output  PseudoPeriodic=off  Frequencies=[]  VectorFormat=1-D array  Unit=W  AffineConversion=off
  SEHoldNode06HeatFlowSensor : fl_lib/Thermal/Thermal Sensors/Heat Flow Rate Sensor
  SEHoldNode07HeatFlowPS : nesl_utility/PS-Simulink Converter  PhysicalDomain=network_engine_domain  SubClassName=ps_output  LeftPortType=input  RightPortType=output  PseudoPeriodic=off  Frequencies=[]  VectorFormat=1-D array  Unit=W  AffineConversion=off
  SEHoldNode07HeatFlowSensor : fl_lib/Thermal/Thermal Sensors/Heat Flow Rate Sensor
  SEHoldNode08HeatFlowPS : nesl_utility/PS-Simulink Converter  PhysicalDomain=network_engine_domain  SubClassName=ps_output  LeftPortType=input  RightPortType=output  PseudoPeriodic=off  Frequencies=[]  VectorFormat=1-D array  Unit=W  AffineConversion=off
  SEHoldNode08HeatFlowSensor : fl_lib/Thermal/Thermal Sensors/Heat Flow Rate Sensor
  SEHoldNode09HeatFlowPS : nesl_utility/PS-Simulink Converter  PhysicalDomain=network_engine_domain  SubClassName=ps_output  LeftPortType=input  RightPortType=output  PseudoPeriodic=off  Frequencies=[]  VectorFormat=1-D array  Unit=W  AffineConversion=off
  SEHoldNode09HeatFlowSensor : fl_lib/Thermal/Thermal Sensors/Heat Flow Rate Sensor
  SEHoldNode10HeatFlowPS : nesl_utility/PS-Simulink Converter  PhysicalDomain=network_engine_domain  SubClassName=ps_output  LeftPortType=input  RightPortType=output  PseudoPeriodic=off  Frequencies=[]  VectorFormat=1-D array  Unit=W  AffineConversion=off
  SEHoldNode10HeatFlowSensor : fl_lib/Thermal/Thermal Sensors/Heat Flow Rate Sensor
  SEHoldNode11HeatFlowPS : nesl_utility/PS-Simulink Converter  PhysicalDomain=network_engine_domain  SubClassName=ps_output  LeftPortType=input  RightPortType=output  PseudoPeriodic=off  Frequencies=[]  VectorFormat=1-D array  Unit=W  AffineConversion=off
  SEHoldNode11HeatFlowSensor : fl_lib/Thermal/Thermal Sensors/Heat Flow Rate Sensor
  SEHoldNode12HeatFlowPS : nesl_utility/PS-Simulink Converter  PhysicalDomain=network_engine_domain  SubClassName=ps_output  LeftPortType=input  RightPortType=output  PseudoPeriodic=off  Frequencies=[]  VectorFormat=1-D array  Unit=W  AffineConversion=off
  SEHoldNode12HeatFlowSensor : fl_lib/Thermal/Thermal Sensors/Heat Flow Rate Sensor
  SEHoldNode13HeatFlowPS : nesl_utility/PS-Simulink Converter  PhysicalDomain=network_engine_domain  SubClassName=ps_output  LeftPortType=input  RightPortType=output  PseudoPeriodic=off  Frequencies=[]  VectorFormat=1-D array  Unit=W  AffineConversion=off
  SEHoldNode13HeatFlowSensor : fl_lib/Thermal/Thermal Sensors/Heat Flow Rate Sensor
  SEHoldNode14HeatFlowPS : nesl_utility/PS-Simulink Converter  PhysicalDomain=network_engine_domain  SubClassName=ps_output  LeftPortType=input  RightPortType=output  PseudoPeriodic=off  Frequencies=[]  VectorFormat=1-D array  Unit=W  AffineConversion=off
  SEHoldNode14HeatFlowSensor : fl_lib/Thermal/Thermal Sensors/Heat Flow Rate Sensor
  SEHoldNode15HeatFlowPS : nesl_utility/PS-Simulink Converter  PhysicalDomain=network_engine_domain  SubClassName=ps_output  LeftPortType=input  RightPortType=output  PseudoPeriodic=off  Frequencies=[]  VectorFormat=1-D array  Unit=W  AffineConversion=off
  SEHoldNode15HeatFlowSensor : fl_lib/Thermal/Thermal Sensors/Heat Flow Rate Sensor
  SEHoldNode16HeatFlowPS : nesl_utility/PS-Simulink Converter  PhysicalDomain=network_engine_domain  SubClassName=ps_output  LeftPortType=input  RightPortType=output  PseudoPeriodic=off  Frequencies=[]  VectorFormat=1-D array  Unit=W  AffineConversion=off
  SEHoldNode16HeatFlowSensor : fl_lib/Thermal/Thermal Sensors/Heat Flow Rate Sensor
  SEHoldNode17HeatFlowPS : nesl_utility/PS-Simulink Converter  PhysicalDomain=network_engine_domain  SubClassName=ps_output  LeftPortType=input  RightPortType=output  PseudoPeriodic=off  Frequencies=[]  VectorFormat=1-D array  Unit=W  AffineConversion=off
  SEHoldNode17HeatFlowSensor : fl_lib/Thermal/Thermal Sensors/Heat Flow Rate Sensor
  SEHoldNode18HeatFlowPS : nesl_utility/PS-Simulink Converter  PhysicalDomain=network_engine_domain  SubClassName=ps_output  LeftPortType=input  RightPortType=output  PseudoPeriodic=off  Frequencies=[]  VectorFormat=1-D array  Unit=W  AffineConversion=off
  SEHoldNode18HeatFlowSensor : fl_lib/Thermal/Thermal Sensors/Heat Flow Rate Sensor
  SEHoldNode19HeatFlowPS : nesl_utility/PS-Simulink Converter  PhysicalDomain=network_engine_domain  SubClassName=ps_output  LeftPortType=input  RightPortType=output  PseudoPeriodic=off  Frequencies=[]  VectorFormat=1-D array  Unit=W  AffineConversion=off
  SEHoldNode19HeatFlowSensor : fl_lib/Thermal/Thermal Sensors/Heat Flow Rate Sensor
  SEHoldNode20HeatFlowPS : nesl_utility/PS-Simulink Converter  PhysicalDomain=network_engine_domain  SubClassName=ps_output  LeftPortType=input  RightPortType=output  PseudoPeriodic=off  Frequencies=[]  VectorFormat=1-D array  Unit=W  AffineConversion=off
  SEHoldNode20HeatFlowSensor : fl_lib/Thermal/Thermal Sensors/Heat Flow Rate Sensor
  SEHoldNode21HeatFlowPS : nesl_utility/PS-Simulink Converter  PhysicalDomain=network_engine_domain  SubClassName=ps_output  LeftPortType=input  RightPortType=output  PseudoPeriodic=off  Frequencies=[]  VectorFormat=1-D array  Unit=W  AffineConversion=off
  SEHoldNode21HeatFlowSensor : fl_lib/Thermal/Thermal Sensors/Heat Flow Rate Sensor
  SharedSEColdEndJunction : SimscapeFluids_lib/Thermal Liquid/Pipes & Fittings/T-Junction (TL)  area_main=se_article_pipe_fa m^2  area_branch=se_article_pipe_fa m^2  junction_spec=fluids.thermal_liquid.pipes_fittings.enum.TLossCoefficientModel.Crane  k_main_converge=1.12  k_main_diverge=1.12  k_branch_converge=1.12  k_branch_diverge=1.12  loss_coeff_A=1  loss_coeff_B=1  loss_coeff_C=1  radius=0.001 m  Re_c=150  Re_0=10  tau=0.0001 s  saturation_ratio=0.2  smoothing_factor=0.01  inertia=false
      settings: InternalSimscapePortConfiguration="{\"Bottom\":[{\"id\":\"C\",\"label\":\"C\",\"type\":\"foundation.thermal_liquid.thermal_liquid\"}],\"Left\":[{\"id\":\"A\",\"label\":\"A\",\"type\":\"foundation.thermal_liquid.thermal_liquid\"}],\"Right\":[{\"id\":\"B\",\"label\":\"B\",\"type\":\"foundation.thermal_liquid.thermal_liquid\"}],\"Top\":[]}"
  SharedSEHotEndJunction : SimscapeFluids_lib/Thermal Liquid/Pipes & Fittings/T-Junction (TL)  area_main=se_article_pipe_fa m^2  area_branch=se_article_pipe_fa m^2  junction_spec=fluids.thermal_liquid.pipes_fittings.enum.TLossCoefficientModel.Crane  k_main_converge=1.12  k_main_diverge=1.12  k_branch_converge=1.12  k_branch_diverge=1.12  loss_coeff_A=1  loss_coeff_B=1  loss_coeff_C=1  radius=0.001 m  Re_c=150  Re_0=10  tau=0.0001 s  saturation_ratio=0.2  smoothing_factor=0.01  inertia=false
      settings: InternalSimscapePortConfiguration="{\"Bottom\":[{\"id\":\"C\",\"label\":\"C\",\"type\":\"foundation.thermal_liquid.thermal_liquid\"}],\"Left\":[{\"id\":\"A\",\"label\":\"A\",\"type\":\"foundation.thermal_liquid.thermal_liquid\"}],\"Right\":[{\"id\":\"B\",\"label\":\"B\",\"type\":\"foundation.thermal_liquid.thermal_liquid\"}],\"Top\":[]}"
  Subsystem2 : Subsystem
  ToWorkspace_se_hold_node01_heatflow_W : ToWorkspace  VariableName=se_hold_node01_heatflow_W  SaveFormat=Structure With Time  SampleTime=-1
  ToWorkspace_se_hold_node02_heatflow_W : ToWorkspace  VariableName=se_hold_node02_heatflow_W  SaveFormat=Structure With Time  SampleTime=-1
  ToWorkspace_se_hold_node03_heatflow_W : ToWorkspace  VariableName=se_hold_node03_heatflow_W  SaveFormat=Structure With Time  SampleTime=-1
  ToWorkspace_se_hold_node04_heatflow_W : ToWorkspace  VariableName=se_hold_node04_heatflow_W  SaveFormat=Structure With Time  SampleTime=-1
  ToWorkspace_se_hold_node05_heatflow_W : ToWorkspace  VariableName=se_hold_node05_heatflow_W  SaveFormat=Structure With Time  SampleTime=-1
  ToWorkspace_se_hold_node06_heatflow_W : ToWorkspace  VariableName=se_hold_node06_heatflow_W  SaveFormat=Structure With Time  SampleTime=-1
  ToWorkspace_se_hold_node07_heatflow_W : ToWorkspace  VariableName=se_hold_node07_heatflow_W  SaveFormat=Structure With Time  SampleTime=-1
  ToWorkspace_se_hold_node08_heatflow_W : ToWorkspace  VariableName=se_hold_node08_heatflow_W  SaveFormat=Structure With Time  SampleTime=-1
  ToWorkspace_se_hold_node09_heatflow_W : ToWorkspace  VariableName=se_hold_node09_heatflow_W  SaveFormat=Structure With Time  SampleTime=-1
  ToWorkspace_se_hold_node10_heatflow_W : ToWorkspace  VariableName=se_hold_node10_heatflow_W  SaveFormat=Structure With Time  SampleTime=-1
  ToWorkspace_se_hold_node11_heatflow_W : ToWorkspace  VariableName=se_hold_node11_heatflow_W  SaveFormat=Structure With Time  SampleTime=-1
  ToWorkspace_se_hold_node12_heatflow_W : ToWorkspace  VariableName=se_hold_node12_heatflow_W  SaveFormat=Structure With Time  SampleTime=-1
  ToWorkspace_se_hold_node13_heatflow_W : ToWorkspace  VariableName=se_hold_node13_heatflow_W  SaveFormat=Structure With Time  SampleTime=-1
  ToWorkspace_se_hold_node14_heatflow_W : ToWorkspace  VariableName=se_hold_node14_heatflow_W  SaveFormat=Structure With Time  SampleTime=-1
  ToWorkspace_se_hold_node15_heatflow_W : ToWorkspace  VariableName=se_hold_node15_heatflow_W  SaveFormat=Structure With Time  SampleTime=-1
  ToWorkspace_se_hold_node16_heatflow_W : ToWorkspace  VariableName=se_hold_node16_heatflow_W  SaveFormat=Structure With Time  SampleTime=-1
  ToWorkspace_se_hold_node17_heatflow_W : ToWorkspace  VariableName=se_hold_node17_heatflow_W  SaveFormat=Structure With Time  SampleTime=-1
  ToWorkspace_se_hold_node18_heatflow_W : ToWorkspace  VariableName=se_hold_node18_heatflow_W  SaveFormat=Structure With Time  SampleTime=-1
  ToWorkspace_se_hold_node19_heatflow_W : ToWorkspace  VariableName=se_hold_node19_heatflow_W  SaveFormat=Structure With Time  SampleTime=-1
  ToWorkspace_se_hold_node20_heatflow_W : ToWorkspace  VariableName=se_hold_node20_heatflow_W  SaveFormat=Structure With Time  SampleTime=-1
  ToWorkspace_se_hold_node21_heatflow_W : ToWorkspace  VariableName=se_hold_node21_heatflow_W  SaveFormat=Structure With Time  SampleTime=-1
  Conn1 : PMIOPort  Side=Left
  Conn2 : PMIOPort  Port=2  Side=Left
  Conn3 : PMIOPort  Port=3  Side=Left
  Conn4 : PMIOPort  Port=4  Side=Left
  NodeTemp21Out : Outport
  wires:
  ConstitutiveHeat21_W/1 -> Subsystem2/1(ConstitutiveHeat21_W)
  Subsystem2/1(NodeTemp21Out) -> NodeTemp21Out/1
  HoldThermalGateCommandFromWorkspace/1 -> HoldThermalGateCommandPS/1
  SEHoldNode01HeatFlowPS/1 -> ToWorkspace_se_hold_node01_heatflow_W/1
  SEHoldNode02HeatFlowPS/1 -> ToWorkspace_se_hold_node02_heatflow_W/1
  SEHoldNode03HeatFlowPS/1 -> ToWorkspace_se_hold_node03_heatflow_W/1
  SEHoldNode04HeatFlowPS/1 -> ToWorkspace_se_hold_node04_heatflow_W/1
  SEHoldNode05HeatFlowPS/1 -> ToWorkspace_se_hold_node05_heatflow_W/1
  SEHoldNode06HeatFlowPS/1 -> ToWorkspace_se_hold_node06_heatflow_W/1
  SEHoldNode07HeatFlowPS/1 -> ToWorkspace_se_hold_node07_heatflow_W/1
  SEHoldNode08HeatFlowPS/1 -> ToWorkspace_se_hold_node08_heatflow_W/1
  SEHoldNode09HeatFlowPS/1 -> ToWorkspace_se_hold_node09_heatflow_W/1
  SEHoldNode10HeatFlowPS/1 -> ToWorkspace_se_hold_node10_heatflow_W/1
  SEHoldNode11HeatFlowPS/1 -> ToWorkspace_se_hold_node11_heatflow_W/1
  SEHoldNode12HeatFlowPS/1 -> ToWorkspace_se_hold_node12_heatflow_W/1
  SEHoldNode13HeatFlowPS/1 -> ToWorkspace_se_hold_node13_heatflow_W/1
  SEHoldNode14HeatFlowPS/1 -> ToWorkspace_se_hold_node14_heatflow_W/1
  SEHoldNode15HeatFlowPS/1 -> ToWorkspace_se_hold_node15_heatflow_W/1
  SEHoldNode16HeatFlowPS/1 -> ToWorkspace_se_hold_node16_heatflow_W/1
  SEHoldNode17HeatFlowPS/1 -> ToWorkspace_se_hold_node17_heatflow_W/1
  SEHoldNode18HeatFlowPS/1 -> ToWorkspace_se_hold_node18_heatflow_W/1
  SEHoldNode19HeatFlowPS/1 -> ToWorkspace_se_hold_node19_heatflow_W/1
  SEHoldNode20HeatFlowPS/1 -> ToWorkspace_se_hold_node20_heatflow_W/1
  SEHoldNode21HeatFlowPS/1 -> ToWorkspace_se_hold_node21_heatflow_W/1
  connections:
  HoldPipe_001/LConn2 -- HoldThermalGate_001/LConn1
  HoldPipe_002/LConn2 -- HoldThermalGate_002/LConn1
  HoldPipe_003/LConn2 -- HoldThermalGate_003/LConn1
  HoldPipe_004/LConn2 -- HoldThermalGate_004/LConn1
  HoldPipe_005/LConn2 -- HoldThermalGate_005/LConn1
  HoldPipe_006/LConn2 -- HoldThermalGate_006/LConn1
  HoldPipe_007/LConn2 -- HoldThermalGate_007/LConn1
  HoldPipe_008/LConn2 -- HoldThermalGate_008/LConn1
  HoldPipe_009/LConn2 -- HoldThermalGate_009/LConn1
  HoldPipe_010/LConn2 -- HoldThermalGate_010/LConn1
  HoldPipe_011/LConn2 -- HoldThermalGate_011/LConn1
  HoldPipe_012/LConn2 -- HoldThermalGate_012/LConn1
  HoldPipe_013/LConn2 -- HoldThermalGate_013/LConn1
  HoldPipe_014/LConn2 -- HoldThermalGate_014/LConn1
  HoldPipe_015/LConn2 -- HoldThermalGate_015/LConn1
  HoldPipe_016/LConn2 -- HoldThermalGate_016/LConn1
  HoldPipe_017/LConn2 -- HoldThermalGate_017/LConn1
  HoldPipe_018/LConn2 -- HoldThermalGate_018/LConn1
  HoldPipe_019/LConn2 -- HoldThermalGate_019/LConn1
  HoldPipe_020/LConn2 -- HoldThermalGate_020/LConn1
  HoldPipe_021/LConn2 -- HoldThermalGate_021/LConn1
  HoldPipe_021/LConn1 -- HoldPipe_020/RConn1
  HoldPipe_020/LConn1 -- HoldPipe_019/RConn1
  HoldPipe_019/LConn1 -- HoldPipe_018/RConn1
  HoldPipe_018/LConn1 -- HoldPipe_017/RConn1
  HoldPipe_017/LConn1 -- HoldPipe_016/RConn1
  HoldPipe_016/LConn1 -- HoldPipe_015/RConn1
  HoldPipe_015/LConn1 -- HoldPipe_014/RConn1
  HoldPipe_014/LConn1 -- HoldPipe_013/RConn1
  HoldPipe_013/LConn1 -- HoldPipe_012/RConn1
  HoldPipe_012/LConn1 -- HoldPipe_011/RConn1
  HoldPipe_011/LConn1 -- HoldPipe_010/RConn1
  HoldPipe_010/LConn1 -- HoldPipe_009/RConn1
  HoldPipe_009/LConn1 -- HoldPipe_008/RConn1
  HoldPipe_008/LConn1 -- HoldPipe_007/RConn1
  HoldPipe_007/LConn1 -- HoldPipe_006/RConn1
  HoldPipe_006/LConn1 -- HoldPipe_005/RConn1
  HoldPipe_005/LConn1 -- HoldPipe_004/RConn1
  HoldPipe_004/LConn1 -- HoldPipe_003/RConn1
  HoldPipe_003/LConn1 -- HoldPipe_002/RConn1
  HoldPipe_002/LConn1 -- HoldPipe_001/RConn1
  HoldThermalGateCommandPS/RConn1 -- HoldThermalGate_001/LConn2 -- HoldThermalGate_002/LConn2 -- HoldThermalGate_003/LConn2 -- HoldThermalGate_004/LConn2 -- HoldThermalGate_005/LConn2 -- HoldThermalGate_006/LConn2 -- HoldThermalGate_007/LConn2 -- HoldThermalGate_008/LConn2 -- HoldThermalGate_009/LConn2 -- HoldThermalGate_010/LConn2 -- HoldThermalGate_011/LConn2 -- HoldThermalGate_012/LConn2 -- HoldThermalGate_013/LConn2 -- HoldThermalGate_014/LConn2 -- HoldThermalGate_015/LConn2 -- HoldThermalGate_016/LConn2 -- HoldThermalGate_017/LConn2 -- HoldThermalGate_018/LConn2 -- HoldThermalGate_019/LConn2 -- HoldThermalGate_020/LConn2 -- HoldThermalGate_021/LConn2
  HoldPipe_001/LConn1 -- SharedSEHotEndJunction/LConn1
  Conn2/RConn1 -- SharedSEHotEndJunction/RConn1
  Conn3/RConn1 -- SharedSEHotEndJunction/RConn2
  HoldPipe_021/RConn1 -- SharedSEColdEndJunction/LConn1
  Conn1/RConn1 -- SharedSEColdEndJunction/RConn1
  Conn4/RConn1 -- SharedSEColdEndJunction/RConn2
  HoldThermalGate_001/RConn1 -- SEHoldNode01HeatFlowSensor/LConn1
  SEHoldNode01HeatFlowSensor/RConn2 -- Subsystem2/RConn1
  SEHoldNode01HeatFlowSensor/RConn1 -- SEHoldNode01HeatFlowPS/LConn1
  HoldThermalGate_002/RConn1 -- SEHoldNode02HeatFlowSensor/LConn1
  SEHoldNode02HeatFlowSensor/RConn2 -- Subsystem2/RConn2
  SEHoldNode02HeatFlowSensor/RConn1 -- SEHoldNode02HeatFlowPS/LConn1
  HoldThermalGate_003/RConn1 -- SEHoldNode03HeatFlowSensor/LConn1
  SEHoldNode03HeatFlowSensor/RConn2 -- Subsystem2/RConn3
  SEHoldNode03HeatFlowSensor/RConn1 -- SEHoldNode03HeatFlowPS/LConn1
  HoldThermalGate_004/RConn1 -- SEHoldNode04HeatFlowSensor/LConn1
  SEHoldNode04HeatFlowSensor/RConn2 -- Subsystem2/RConn4
  SEHoldNode04HeatFlowSensor/RConn1 -- SEHoldNode04HeatFlowPS/LConn1
  HoldThermalGate_005/RConn1 -- SEHoldNode05HeatFlowSensor/LConn1
  SEHoldNode05HeatFlowSensor/RConn2 -- Subsystem2/RConn5
  SEHoldNode05HeatFlowSensor/RConn1 -- SEHoldNode05HeatFlowPS/LConn1
  HoldThermalGate_006/RConn1 -- SEHoldNode06HeatFlowSensor/LConn1
  SEHoldNode06HeatFlowSensor/RConn2 -- Subsystem2/RConn6
  SEHoldNode06HeatFlowSensor/RConn1 -- SEHoldNode06HeatFlowPS/LConn1
  HoldThermalGate_007/RConn1 -- SEHoldNode07HeatFlowSensor/LConn1
  SEHoldNode07HeatFlowSensor/RConn2 -- Subsystem2/RConn7
  SEHoldNode07HeatFlowSensor/RConn1 -- SEHoldNode07HeatFlowPS/LConn1
  HoldThermalGate_008/RConn1 -- SEHoldNode08HeatFlowSensor/LConn1
  SEHoldNode08HeatFlowSensor/RConn2 -- Subsystem2/RConn8
  SEHoldNode08HeatFlowSensor/RConn1 -- SEHoldNode08HeatFlowPS/LConn1
  HoldThermalGate_009/RConn1 -- SEHoldNode09HeatFlowSensor/LConn1
  SEHoldNode09HeatFlowSensor/RConn2 -- Subsystem2/RConn9
  SEHoldNode09HeatFlowSensor/RConn1 -- SEHoldNode09HeatFlowPS/LConn1
  HoldThermalGate_010/RConn1 -- SEHoldNode10HeatFlowSensor/LConn1
  SEHoldNode10HeatFlowSensor/RConn2 -- Subsystem2/RConn10
  SEHoldNode10HeatFlowSensor/RConn1 -- SEHoldNode10HeatFlowPS/LConn1
  HoldThermalGate_011/RConn1 -- SEHoldNode11HeatFlowSensor/LConn1
  SEHoldNode11HeatFlowSensor/RConn2 -- Subsystem2/RConn11
  SEHoldNode11HeatFlowSensor/RConn1 -- SEHoldNode11HeatFlowPS/LConn1
  HoldThermalGate_012/RConn1 -- SEHoldNode12HeatFlowSensor/LConn1
  SEHoldNode12HeatFlowSensor/RConn2 -- Subsystem2/RConn12
  SEHoldNode12HeatFlowSensor/RConn1 -- SEHoldNode12HeatFlowPS/LConn1
  HoldThermalGate_013/RConn1 -- SEHoldNode13HeatFlowSensor/LConn1
  SEHoldNode13HeatFlowSensor/RConn2 -- Subsystem2/RConn13
  SEHoldNode13HeatFlowSensor/RConn1 -- SEHoldNode13HeatFlowPS/LConn1
  HoldThermalGate_014/RConn1 -- SEHoldNode14HeatFlowSensor/LConn1
  SEHoldNode14HeatFlowSensor/RConn2 -- Subsystem2/RConn14
  SEHoldNode14HeatFlowSensor/RConn1 -- SEHoldNode14HeatFlowPS/LConn1
  HoldThermalGate_015/RConn1 -- SEHoldNode15HeatFlowSensor/LConn1
  SEHoldNode15HeatFlowSensor/RConn2 -- Subsystem2/RConn15
  SEHoldNode15HeatFlowSensor/RConn1 -- SEHoldNode15HeatFlowPS/LConn1
  HoldThermalGate_016/RConn1 -- SEHoldNode16HeatFlowSensor/LConn1
  SEHoldNode16HeatFlowSensor/RConn2 -- Subsystem2/RConn16
  SEHoldNode16HeatFlowSensor/RConn1 -- SEHoldNode16HeatFlowPS/LConn1
  HoldThermalGate_017/RConn1 -- SEHoldNode17HeatFlowSensor/LConn1
  SEHoldNode17HeatFlowSensor/RConn2 -- Subsystem2/RConn17
  SEHoldNode17HeatFlowSensor/RConn1 -- SEHoldNode17HeatFlowPS/LConn1
  HoldThermalGate_018/RConn1 -- SEHoldNode18HeatFlowSensor/LConn1
  SEHoldNode18HeatFlowSensor/RConn2 -- Subsystem2/RConn18
  SEHoldNode18HeatFlowSensor/RConn1 -- SEHoldNode18HeatFlowPS/LConn1
  HoldThermalGate_019/RConn1 -- SEHoldNode19HeatFlowSensor/LConn1
  SEHoldNode19HeatFlowSensor/RConn2 -- Subsystem2/RConn19
  SEHoldNode19HeatFlowSensor/RConn1 -- SEHoldNode19HeatFlowPS/LConn1
  HoldThermalGate_020/RConn1 -- SEHoldNode20HeatFlowSensor/LConn1
  SEHoldNode20HeatFlowSensor/RConn2 -- Subsystem2/RConn20
  SEHoldNode20HeatFlowSensor/RConn1 -- SEHoldNode20HeatFlowPS/LConn1
  HoldThermalGate_021/RConn1 -- SEHoldNode21HeatFlowSensor/LConn1
  SEHoldNode21HeatFlowSensor/RConn2 -- Subsystem2/RConn21
  SEHoldNode21HeatFlowSensor/RConn1 -- SEHoldNode21HeatFlowPS/LConn1
